simulink model "structure_lofi"  (R2026b)
settings: Solver=VariableStepAuto
undefined symbols (not defined in the file or in its folder): DiscIntNeverNeededParam, P, Ts
libraries: fl_lib x14, nesl_utility x10, simulink x5, robotmobilelib x1
settings Model: Creator=aomar  LastModifiedBy=aomar

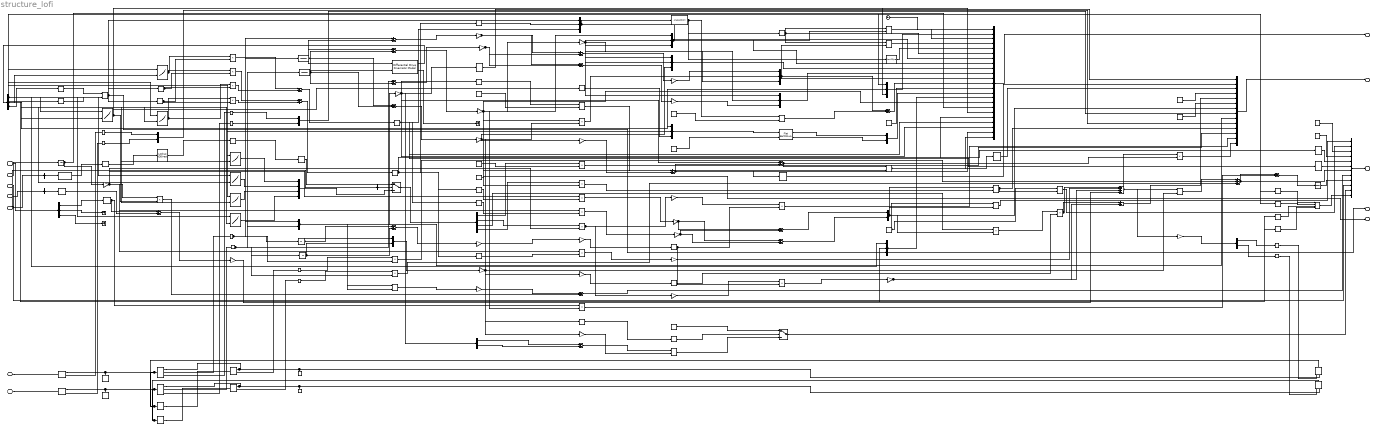
== system structure_lofi ==
  wrench : Inport
  dmdt : Inport  Port=2
  E_impl : Inport  Port=3
  env_dist : Inport  Port=4  OutDataTypeStr=Bus: Bus_EnvDisturbance
  env_ovr : Inport  Port=5  OutDataTypeStr=Bus: Bus_EnvOverride
  Br : Gain  Gain=P.structure.geom.B
  Clock : Clock
  DCM_WB : Angle2Dcm
      settings: AttributesFormatString=Rotation Order: %<rotationOrder>
  DDKM : robotmobilelib/Differential Drive Kinematic Model  VehicleInputs=Wheel Speeds  WheelRadius=P.structure.r_sprocket*(1-P.structure.lofi.i_nom)  WheelSpeedRange=[-inf inf]  TrackWidth=P.structure.lofi.chi*P.structure.geom.B  InitialState=P.structure.init.pose2D0(:)  SimulateUsing=Code generation
  D_R : UnaryMinus
  Dist : BusSelector  OutputSignals=F_ext_B
  E_diss_J : DiscreteIntegrator  gainval=1  SampleTime=Ts.base  ICPrevOutput=DiscIntNeverNeededParam  ICPrevScaledInput=DiscIntNeverNeededParam
  E_kin : Gain  Gain=0.5*P.structure.lofi.J_side
  E_mech : Sum
  E_pot : Product  Inputs=**
  F_diss : Sum
  F_grade : Gain  Gain=0.5
  F_load : Sum  Inputs=+++-
  F_push : Sum
  F_roll : Product  Inputs=**
  F_turn : Product  Inputs=**
  Fext_x : Selector  InputPortWidth=3  IndexOptions=Index vector (dialog)  Indices=1  OutputSizes=1
  Fimpl_x : Selector  InputPortWidth=3  IndexOptions=Index vector (dialog)  Indices=1  OutputSizes=1
  Flat_Earth_to_LLA : FlatEarth2LLA  LL0=P.world.lla0(1:2)
  Fric_Sensor_L : fl_lib/Mechanical/Mechanical Sensors/Ideal Torque Sensor
  Fric_Sensor_R : fl_lib/Mechanical/Mechanical Sensors/Ideal Torque Sensor
  Friction_L : fl_lib/Mechanical/Rotational Elements/Rotational Friction  brkwy_trq=P.structure.track.T_brk N*m  brkwy_vel=P.structure.track.w_brk rad/s  Col_trq=P.structure.track.T_col N*m  visc_coef=P.structure.track.c_visc N*m*s/rad  w_specify=off  w_priority=None  w=0 rad/s  w_nominal_specify=off  w_nominal_value=1  w_nominal_unit=rad/s  t_specify=off  t_priority=None  t=0 N*m  t_nominal_specify=off  t_nominal_value=1  t_nominal_unit=N*m
  Friction_R : fl_lib/Mechanical/Rotational Elements/Rotational Friction  brkwy_trq=P.structure.track.T_brk N*m  brkwy_vel=P.structure.track.w_brk rad/s  Col_trq=P.structure.track.T_col N*m  visc_coef=P.structure.track.c_visc N*m*s/rad  w_specify=off  w_priority=None  w=0 rad/s  w_nominal_specify=off  w_nominal_value=1  w_nominal_unit=rad/s  t_specify=off  t_priority=None  t=0 N*m  t_nominal_specify=off  t_nominal_value=1  t_nominal_unit=N*m
  H : Lookup_n-D  BreakpointsForDimension1=P.world.terrain.xE  BreakpointsForDimension2=P.world.terrain.yN  IndexSearchMethod=Evenly spaced points  Table=P.world.terrain.H  ExtrapMethod=Clip  InternalRulePriority=Speed  RndMeth=Simplest
      settings: InputPortMap=u0,u1
  J_side_L : fl_lib/Mechanical/Rotational Elements/Inertia  inertia=P.structure.lofi.J_side kg*m^2  num_ports=foundation.enum.numPorts2.one  w_specify=on  w_priority=High  w=P.structure.init.v0/P.structure.r_sprocket rad/s  w_nominal_specify=off  w_nominal_value=1  w_nominal_unit=rad/s  t_specify=off  t_priority=None  t=0 N*m  t_nominal_specify=off  t_nominal_value=1  t_nominal_unit=N*m
  J_side_R : fl_lib/Mechanical/Rotational Elements/Inertia  inertia=P.structure.lofi.J_side kg*m^2  num_ports=foundation.enum.numPorts2.one  w_specify=on  w_priority=High  w=P.structure.init.v0/P.structure.r_sprocket rad/s  w_nominal_specify=off  w_nominal_value=1  w_nominal_unit=rad/s  t_specify=off  t_priority=None  t=0 N*m  t_nominal_specify=off  t_nominal_value=1  t_nominal_unit=N*m
  Load_Torque_L : fl_lib/Mechanical/Mechanical Sources/Ideal Torque Source
  Load_Torque_R : fl_lib/Mechanical/Mechanical Sources/Ideal Torque Source
  Mass : Integrator  InitialCondition=P.structure.mp.m0
  Motion_Sensor_L : fl_lib/Mechanical/Mechanical Sensors/Ideal Rotational Motion Sensor  reference=foundation.enum.MeasurementReference.difference  acceleration_port=false  velocity_port=true  position_port=true  wrap_angle=false  offset=0 rad
  Motion_Sensor_R : fl_lib/Mechanical/Mechanical Sensors/Ideal Rotational Motion Sensor  reference=foundation.enum.MeasurementReference.difference  acceleration_port=false  velocity_port=true  position_port=true  wrap_angle=false  offset=0 rad
  Mres : Gain  Gain=-P.structure.geom.L/4
  Mturn : Product  Inputs=**
  N_L : Sum  Inputs=+-
  N_LR : Mux  Inputs=2
  N_R : Sum
  N_pt : Product  Inputs=**  Multiplication=Matrix(*)
  NaN : Constant  Value=NaN  VectorParams1D=off
  Ones2 : Constant  Value=ones(2,1)  VectorParams1D=off
  Out_of_map : Logic  Operator=OR  Inputs=4  AllPortsSameDT=off  OutDataTypeStr=boolean
  Ovr_soil_id : BusSelector  OutputSignals=soil_id
  Ovr_use_soil : BusSelector  OutputSignals=use_soil
  PSS_T_L : nesl_utility/PS-Simulink Converter  PhysicalDomain=network_engine_domain  SubClassName=ps_output  LeftPortType=input  RightPortType=output  PseudoPeriodic=off  Frequencies=[]  VectorFormat=inherit  Unit=N*m  AffineConversion=off
  PSS_T_R : nesl_utility/PS-Simulink Converter  PhysicalDomain=network_engine_domain  SubClassName=ps_output  LeftPortType=input  RightPortType=output  PseudoPeriodic=off  Frequencies=[]  VectorFormat=inherit  Unit=N*m  AffineConversion=off
  PSS_Tf_L : nesl_utility/PS-Simulink Converter  PhysicalDomain=network_engine_domain  SubClassName=ps_output  LeftPortType=input  RightPortType=output  PseudoPeriodic=off  Frequencies=[]  VectorFormat=inherit  Unit=N*m  AffineConversion=off
  PSS_Tf_R : nesl_utility/PS-Simulink Converter  PhysicalDomain=network_engine_domain  SubClassName=ps_output  LeftPortType=input  RightPortType=output  PseudoPeriodic=off  Frequencies=[]  VectorFormat=inherit  Unit=N*m  AffineConversion=off
  PSS_th_L : nesl_utility/PS-Simulink Converter  PhysicalDomain=network_engine_domain  SubClassName=ps_output  LeftPortType=input  RightPortType=output  PseudoPeriodic=off  Frequencies=[]  VectorFormat=inherit  Unit=rad  AffineConversion=off
  PSS_th_R : nesl_utility/PS-Simulink Converter  PhysicalDomain=network_engine_domain  SubClassName=ps_output  LeftPortType=input  RightPortType=output  PseudoPeriodic=off  Frequencies=[]  VectorFormat=inherit  Unit=rad  AffineConversion=off
  PSS_w_L : nesl_utility/PS-Simulink Converter  PhysicalDomain=network_engine_domain  SubClassName=ps_output  LeftPortType=input  RightPortType=output  PseudoPeriodic=off  Frequencies=[]  VectorFormat=inherit  Unit=rad/s  AffineConversion=off
  PSS_w_R : nesl_utility/PS-Simulink Converter  PhysicalDomain=network_engine_domain  SubClassName=ps_output  LeftPortType=input  RightPortType=output  PseudoPeriodic=off  Frequencies=[]  VectorFormat=inherit  Unit=rad/s  AffineConversion=off
  P_diss : Sum  Inputs=+++
  P_diss_E : Sum  Inputs=+-
  P_impl : Product  Inputs=**
  P_res : DotProduct  OutDataTypeStr=Inherit: Inherit via internal rule
  Pf_L : Product  Inputs=**
  Pf_R : Product  Inputs=**
  Pslip : Product  Inputs=**
  R_WB : Math  Operator=transpose
  Ref_L : fl_lib/Mechanical/Rotational Elements/Mechanical Rotational Reference
  Ref_R : fl_lib/Mechanical/Rotational Elements/Mechanical Rotational Reference
  SPS_load_L : nesl_utility/Simulink-PS Converter  PhysicalDomain=network_engine_domain  SubClassName=ps_input  LeftPortType=input  RightPortType=output  PseudoPeriodic=off  Frequencies=[]  NoiseDistribution=none  NoiseParameters=[]  Unit=N*m  AffineConversion=off  FilteringAndDerivatives=zero  SimscapeFilterOrder=1  InputFilterTimeConstant=0.001  UdotUserProvided=0
  SPS_load_R : nesl_utility/Simulink-PS Converter  PhysicalDomain=network_engine_domain  SubClassName=ps_input  LeftPortType=input  RightPortType=output  PseudoPeriodic=off  Frequencies=[]  NoiseDistribution=none  NoiseParameters=[]  Unit=N*m  AffineConversion=off  FilteringAndDerivatives=zero  SimscapeFilterOrder=1  InputFilterTimeConstant=0.001  UdotUserProvided=0
  Soil : Demux
  Soil_map : Mux
  Soil_props : Selector  InputPortWidth=6  IndexOptions=Index vector (dialog)  Indices=[2 4 5 6]  OutputSizes=1
  Soil_row : Reshape
  Soil_sw : Switch  Criteria=u2 ~= 0  SaturateOnIntegerOverflow=off  InputSameDT=off
  Soil_table : LookupNDDirect  InputsSelectThisObjectFromTable=Vector  Table=P.world.soilTable'  DiagnosticForOutOfRangeInput=None
  Spread : Constant  Value=kron(eye(2),ones(P.structure.track.Nc,1))  VectorParams1D=off
  State : Demux  Outputs=3
  StructureDiag : BusCreator  Inputs=12  OutDataTypeStr=Bus: Bus_StructureDiag  NonVirtualBus=on
  T_load : Gain  Gain=-P.structure.r_sprocket
  T_load_LR : Demux  Outputs=2
  Term_Mimpl : Terminator
  Term_rimpl : Terminator
  Term_stateDot : Terminator
  Torque_Sensor_L : fl_lib/Mechanical/Mechanical Sensors/Ideal Torque Sensor
  Torque_Sensor_R : fl_lib/Mechanical/Mechanical Sensors/Ideal Torque Sensor
  TrackState : BusCreator  Inputs=14  OutDataTypeStr=Bus: Bus_TrackState  NonVirtualBus=on
  TruthState : BusCreator  Inputs=23  OutDataTypeStr=Bus: Bus_TruthState  NonVirtualBus=on
  Wcos : Product  Inputs=**
  Weight : Gain  Gain=P.frames.g
  Wrench : Demux  Outputs=[3 3 3]
  Wsin_l : Product  Inputs=**
  Wsin_t : Product  Inputs=**
  Zero : Gain  Gain=0
  Zeros14a : Constant  Value=zeros(2*P.structure.track.Nc,1)  VectorParams1D=off
  Zeros14b : Constant  Value=zeros(2*P.structure.track.Nc,1)  VectorParams1D=off
  Zeros2a : Constant  Value=zeros(2,1)  VectorParams1D=off
  Zeros2b : Constant  Value=zeros(2,1)  VectorParams1D=off
  a_diff : Sum  Inputs=-+
  a_err_L : Sum  Inputs=+-
  a_err_R : Sum  Inputs=+-
  a_sum : Sum
  abs_r : Abs  ZeroCross=off  SaturateOnIntegerOverflow=off
  abs_vB : Abs  ZeroCross=off  SaturateOnIntegerOverflow=off
  acc_B : Mux  Inputs=3
  acc_W : Product  Inputs=**  Multiplication=Matrix(*)
  alpha_B : Mux  Inputs=3
  alpha_L : Gain  Gain=1/P.sim.ssc.tau_filt
  alpha_R : Gain  Gain=1/P.sim.ssc.tau_filt
  chi_eff : Switch  Criteria=u2 ~= 0  SaturateOnIntegerOverflow=off  InputSameDT=off
  chi_raw : Product  Inputs=*/
  cos_gl : Trigonometry  Operator=cos
  cos_psi : Trigonometry  Operator=cos
  cos_th : Trigonometry  Operator=cos
  dvB : Sum  Inputs=-+
  eul : Mux  Inputs=3
  fN : Product  Inputs=**
  fRoll_map : Lookup_n-D  BreakpointsForDimension1=P.world.terrain.xE  BreakpointsForDimension2=P.world.terrain.yN  IndexSearchMethod=Evenly spaced points  Table=P.world.soil.fRoll  ExtrapMethod=Clip  InternalRulePriority=Speed  RndMeth=Simplest
      settings: InputPortMap=u0,u1
  g_B : Product  Inputs=**  Multiplication=Matrix(*)
  g_enu : Constant  Value=[0;0;P.frames.g]  VectorParams1D=off
  grade_lat : Trigonometry  Operator=atan
  grade_long : Trigonometry  Operator=atan
  hE : Lookup_n-D  BreakpointsForDimension1=P.world.terrain.xE  BreakpointsForDimension2=P.world.terrain.yN  IndexSearchMethod=Evenly spaced points  Table=P.world.terrain.dHdE  ExtrapMethod=Clip  InternalRulePriority=Speed  RndMeth=Simplest
      settings: InputPortMap=u0,u1
  hE_c : Product  Inputs=**
  hE_s : Product  Inputs=**
  hN : Lookup_n-D  BreakpointsForDimension1=P.world.terrain.xE  BreakpointsForDimension2=P.world.terrain.yN  IndexSearchMethod=Evenly spaced points  Table=P.world.terrain.dHdN  ExtrapMethod=Clip  InternalRulePriority=Speed  RndMeth=Simplest
      settings: InputPortMap=u0,u1
  hN_c : Product  Inputs=**
  hN_s : Product  Inputs=**
  half : Gain  Gain=0.5
  half_B : Gain  Gain=[-1;1]*P.structure.geom.B/2
  half_push : Gain  Gain=0.5
  href : Constant  Value=-P.world.lla0(3)  VectorParams1D=off
  inv_vEps : Gain  Gain=1/P.structure.track.vEpsRR
  inv_wEps : Gain  Gain=1/P.structure.lofi.w_eps
  kN : Product  Inputs=**
  kNc : Constant  Value=P.structure.track.Nc*P.structure.contact.kc  VectorParams1D=off
  kScale_map : Lookup_n-D  BreakpointsForDimension1=P.world.terrain.xE  BreakpointsForDimension2=P.world.terrain.yN  IndexSearchMethod=Evenly spaced points  Table=P.world.soil.kScale  ExtrapMethod=Clip  InternalRulePriority=Speed  RndMeth=Simplest
      settings: InputPortMap=u0,u1
  k_lat : Gain  Gain=P.structure.lofi.h_cg/P.structure.geom.B
  k_turn : Gain  Gain=P.structure.geom.L/(4*P.structure.geom.B)
  kr : Gain  Gain=P.structure.r_sprocket*(1-P.structure.lofi.i_nom)/(P.structure.lofi.chi*P.structure.geom.B)
  kr_d : Gain  Gain=P.structure.r_sprocket*(1-P.structure.lofi.i_nom)/(P.structure.lofi.chi*P.structure.geom.B)
  krd : Gain  Gain=P.structure.r_sprocket*(1-P.structure.lofi.i_nom)/(P.structure.lofi.chi*P.structure.geom.B)
  kv : Gain  Gain=P.structure.r_sprocket*(1-P.structure.lofi.i_nom)/2
  kvd : Gain  Gain=P.structure.r_sprocket*(1-P.structure.lofi.i_nom)/2
  lla : Mux  Inputs=2
  muLat_map : Lookup_n-D  BreakpointsForDimension1=P.world.terrain.xE  BreakpointsForDimension2=P.world.terrain.yN  IndexSearchMethod=Evenly spaced points  Table=P.world.soil.muLat  ExtrapMethod=Clip  InternalRulePriority=Speed  RndMeth=Simplest
      settings: InputPortMap=u0,u1
  muPeak2 : Product  Inputs=**
  muPeak_map : Lookup_n-D  BreakpointsForDimension1=P.world.terrain.xE  BreakpointsForDimension2=P.world.terrain.yN  IndexSearchMethod=Evenly spaced points  Table=P.world.soil.muPeak  ExtrapMethod=Clip  InternalRulePriority=Speed  RndMeth=Simplest
      settings: InputPortMap=u0,u1
  muW : Product  Inputs=**
  omega_B : Mux  Inputs=3
  p_ned : Mux  Inputs=3
  pen_pt : Product  Inputs=**  Multiplication=Matrix(*)
  pos_W : Mux  Inputs=3
  pose2D_mux : Mux  Inputs=3
  psi : Trigonometry  Operator=atan2
  q_WB : Dcm2Quat
  r_cg_B : Constant  Value=P.structure.mp.rcg0_FLU(:)  VectorParams1D=off
  r_small : simulink/Logic and Bit Operations/Compare To Constant  relop=<  const=P.structure.track.chi_rmin  OutDataTypeStr=boolean
  sin_gl : Trigonometry
  sin_gt : Trigonometry
  sin_psi : Trigonometry
  sin_th : Trigonometry
  sink : Product  Inputs=*/
  slip : SignalConversion  OverrideOpt=off
  slip_LR : Product  Inputs=*/
  slopeLat : SignalConversion  OverrideOpt=off
  slopeLong : SignalConversion  OverrideOpt=off
  soil_dbl : DataTypeConversion  OutDataTypeStr=double  SaturateOnIntegerOverflow=off  RndMeth=Floor
  soil_idx0 : Bias  Bias=-1  SaturateOnIntegerOverflow=off
  specForce_B : Sum
  sprAngle : Mux  Inputs=2
  sprTorque : Mux  Inputs=2
  tan_lat : Sum  Inputs=-+
  tan_long : Sum
  tanh_r : Trigonometry  Operator=tanh
  tanh_vb : Trigonometry  Operator=tanh
  theta : UnaryMinus
  turn_sign : Gain  Gain=[-1;1]
  vB_floor : MinMax  Function=max  Inputs=2  ZeroCross=off
  vBelt : Gain  Gain=P.structure.r_sprocket
  vBelt_LR : Demux  Outputs=2
  vGround : Sum
  v_b_d : Gain  Gain=P.structure.r_sprocket
  v_belt : SignalConversion  OverrideOpt=off
  v_eps : Constant  Value=P.structure.track.v_eps_slip  VectorParams1D=off
  v_ground : SignalConversion  OverrideOpt=off
  v_r : Product  Inputs=**
  v_slip : Sum  Inputs=+-
  vel_B : Mux  Inputs=3
  vel_W : Product  Inputs=**  Multiplication=Matrix(*)
  w2J : DotProduct  OutDataTypeStr=Inherit: Inherit via internal rule
  w_d : Mux  Inputs=2
  w_delay_L : UnitDelay  InitialCondition=P.structure.init.v0/P.structure.r_sprocket  SampleTime=Ts.base
  w_delay_R : UnitDelay  InitialCondition=P.structure.init.v0/P.structure.r_sprocket  SampleTime=Ts.base
  w_diff : Sum  Inputs=-+
  w_filt_L : TransferFcn  Numerator=1  Denominator=[P.sim.ssc.tau_filt 1]
  w_filt_R : TransferFcn  Numerator=1  Denominator=[P.sim.ssc.tau_filt 1]
  w_raw : Mux  Inputs=2
  w_sum : Sum
  wd_diff : Sum  Inputs=-+
  x_hi : simulink/Logic and Bit Operations/Compare To Constant  relop=>  const=P.world.terrain.xE(end)  OutDataTypeStr=boolean
  x_lo : simulink/Logic and Bit Operations/Compare To Constant  relop=<  const=P.world.terrain.xE(1)  OutDataTypeStr=boolean
  y_hi : simulink/Logic and Bit Operations/Compare To Constant  relop=>  const=P.world.terrain.yN(end)  OutDataTypeStr=boolean
  y_lo : simulink/Logic and Bit Operations/Compare To Constant  relop=<  const=P.world.terrain.yN(1)  OutDataTypeStr=boolean
  Spr_L : PMIOPort  Side=Left  ConnectionType=Connection: foundation.mechanical.rotational.rotational
  Spr_R : PMIOPort  Port=2  Side=Left  ConnectionType=Connection: foundation.mechanical.rotational.rotational
  truth : Outport  OutDataTypeStr=Bus: Bus_TruthState
  tracks : Outport  Port=2  OutDataTypeStr=Bus: Bus_TrackState
  diag : Outport  Port=3  OutDataTypeStr=Bus: Bus_StructureDiag
  pose2D : Outport  Port=4
  speed_fwd : Outport  Port=5
  wires:
  wrench/1 -> Wrench/1  "wrench"
  dmdt/1 -> Mass/1  "dmdt"
  E_impl/1 -> StructureDiag/10  "E_impl_shaft_J"
  env_dist/1 -> Dist/1  "env_dist"
  env_ovr/1 -> Ovr_soil_id/1, Ovr_use_soil/1  "env_ovr"
  Ovr_soil_id/1 -> soil_dbl/1  "<soil_id>"
  Dist/1 -> Fext_x/1  "<F_ext_B>"
  Wrench/1 -> Fimpl_x/1  "F_impl"
  Wrench/2 -> Term_Mimpl/1  "M_impl"
  Wrench/3 -> Term_rimpl/1  "r_impl"
  sin_th/1 -> psi/1  "sin_th"
  cos_th/1 -> psi/2  "cos_th"
  Mass/1 -> TruthState/17, Weight/1  "mass"
  Fext_x/1 -> F_push/2  "Fext_x"
  soil_dbl/1 -> soil_idx0/1  "soil_dbl"
  PSS_T_L/1 -> sprTorque/1  "T_spr_L"
  PSS_T_R/1 -> sprTorque/2  "T_spr_R"
  psi/1 -> pose2D_mux/3, eul/1, cos_psi/1, sin_psi/1  "psi"
  soil_idx0/1 -> Soil_table/1  "soil_idx0"
  Weight/1 -> Wsin_l/1, muW/2, Wsin_t/1, E_pot/1, Wcos/1  "W"
  Fimpl_x/1 -> P_impl/1, F_push/1  "Fimpl_x"
  H/1 -> E_pot/2, D_R/1, pos_W/3, TruthState/18  "terrainH"
  sprTorque/1 -> TrackState/10  "sprTorque"
  F_push/1 -> half_push/1  "F_push"
  sin_psi/1 -> hE_s/2, hN_s/2  "sin_psi"
  E_pot/1 -> E_mech/2  "E_pot"
  cos_psi/1 -> hE_c/2, hN_c/2  "cos_psi"
  hE/1 -> hE_s/1, hE_c/1  "hE"
  hN/1 -> hN_c/1, hN_s/1  "hN"
  Soil_table/1 -> Soil_row/1  "Soil_table"
  PSS_th_L/1 -> sprAngle/1  "th_L"
  PSS_th_R/1 -> sprAngle/2  "th_R"
  PSS_w_L/1 -> a_err_L/1, w_filt_L/1, Pf_L/2, w_raw/1, w_delay_L/1  "w_L"
  PSS_w_R/1 -> w_filt_R/1, a_err_R/1, Pf_R/2, w_raw/2, w_delay_R/1  "w_R"
  hE_s/1 -> tan_lat/1  "hE_s"
  hE_c/1 -> tan_long/1  "hE_c"
  hN_c/1 -> tan_lat/2  "hN_c"
  hN_s/1 -> tan_long/2  "hN_s"
  Soil_row/1 -> Soil_props/1  "Soil_row"
  half_push/1 -> F_load/4  "F_push_side"
  muPeak_map/1 -> Soil_map/1  "muPeak"
  muLat_map/1 -> Soil_map/2  "muLat"
  fRoll_map/1 -> Soil_map/3  "fRoll"
  kScale_map/1 -> Soil_map/4  "kScale"
  sprAngle/1 -> TrackState/8  "sprAngle"
  Soil_map/1 -> Soil_sw/3  "soil_map"
  w_raw/1 -> vBelt/1, TrackState/9, w2J/2, w2J/1  "sprSpeed"
  PSS_Tf_L/1 -> Pf_L/1  "T_fric_L"
  PSS_Tf_R/1 -> Pf_R/1  "T_fric_R"
  tan_lat/1 -> grade_lat/1  "tan_lat"
  tan_long/1 -> grade_long/1  "tan_long"
  w_delay_L/1 -> wd_diff/1, w_d/1  "w_d_L"
  Soil_props/1 -> Soil_sw/1  "soil_ovr"
  w_delay_R/1 -> wd_diff/2, w_d/2  "w_d_R"
  w_filt_L/1 -> w_diff/1, a_err_L/2, w_sum/1, DDKM/1  "w_L"
  w_filt_R/1 -> w_diff/2, w_sum/2, a_err_R/2, DDKM/2  "w_R"
  Ovr_use_soil/1 -> Soil_sw/2  "<use_soil>"
  w_d/1 -> v_b_d/1  "w_d"
  a_err_L/1 -> alpha_L/1  "a_err_L"
  w_sum/1 -> kv/1  "w_sum"
  a_err_R/1 -> alpha_R/1  "a_err_R"
  w_diff/1 -> kr/1  "w_diff"
  wd_diff/1 -> kr_d/1  "wd_diff"
  grade_long/1 -> theta/1, sin_gl/1, TruthState/19, slopeLong/1, cos_gl/1  "grade_long"
  Pf_L/1 -> P_diss/2  "P_fric_L"
  Pf_R/1 -> P_diss/3  "P_fric_R"
  w2J/1 -> E_kin/1  "w2"
  grade_lat/1 -> eul/3, sin_gt/1, slopeLat/1, TruthState/20  "grade_lat"
  vBelt/1 -> vBelt_LR/1, v_slip/1, TruthState/21, v_belt/1, abs_vB/1  "vBelt_LR"
  Soil_sw/1 -> Soil/1  "soil"
  DDKM/1 -> State/1  "state"
  DDKM/2 -> Term_stateDot/1  "stateDot"
  Soil/1 -> muPeak2/1  "muPeak"
  Soil/2 -> muW/1  "muLat"
  Soil/3 -> fN/1  "fRoll"
  Soil/4 -> kN/1  "kScale"
  vBelt_LR/1 -> dvB/1  "vBelt_L"
  vBelt_LR/2 -> dvB/2  "vBelt_R"
  theta/1 -> eul/2  "theta"
  alpha_L/1 -> a_diff/1, a_sum/1  "alpha_L"
  abs_vB/1 -> vB_floor/1  "abs_vB"
  v_eps/1 -> vB_floor/2  "v_eps"
  kr/1 -> Br/1, abs_r/1, omega_B/3, v_r/2, half_B/1  "r"
  Ones2/1 -> muPeak2/2  "Ones2"
  kNc/1 -> kN/2  "kNc"
  cos_gl/1 -> Wcos/2  "cos_gl"
  sin_gt/1 -> Wsin_t/2  "sin_gt"
  kr_d/1 -> inv_wEps/1  "r_d"
  sin_gl/1 -> Wsin_l/2  "sin_gl"
  E_kin/1 -> E_mech/1  "E_kin"
  v_belt/1 -> TrackState/1  "v_belt"
  kv/1 -> P_impl/2, speed_fwd/1, vel_B/1, Zero/1, vGround/1, v_r/1, TruthState/16  "speed_fwd"
  alpha_R/1 -> a_diff/2, a_sum/2  "alpha_R"
  v_b_d/1 -> P_res/2, inv_vEps/1  "v_b_d"
  eul/1 -> TruthState/7, DCM_WB/1  "eul"
  a_sum/1 -> kvd/1  "a_sum"
  a_diff/1 -> krd/1  "a_diff"
  E_mech/1 -> StructureDiag/8  "E_mech"
  dvB/1 -> chi_raw/1  "dvB"
  Zero/1 -> alpha_B/2, alpha_B/1, acc_B/3, omega_B/2, omega_B/1, vel_B/3, vel_B/2  "Zero"
  D_R/1 -> p_ned/3  "D_R"
  vB_floor/1 -> slip_LR/2  "vB_floor"
  v_r/1 -> acc_B/2  "v_r"
  half_B/1 -> vGround/2  "rB2"
  muPeak2/1 -> TrackState/12  "muPeak"
  kN/1 -> sink/2  "k_track"
  Wcos/1 -> half/1  "Wcos"
  Wsin_t/1 -> k_lat/1  "Wsin_t"
  muW/1 -> k_turn/1, Mres/1  "muLat_W"
  inv_wEps/1 -> tanh_r/1  "inv_wEps"
  Wsin_l/1 -> F_grade/1  "Wsin_l"
  inv_vEps/1 -> tanh_vb/1  "inv_vEps"
  P_impl/1 -> P_diss_E/2  "P_impl_chassis"
  abs_r/1 -> r_small/1  "abs_r"
  Br/1 -> chi_raw/2  "B_r"
  vel_B/1 -> TruthState/8, vel_W/2  "vel_B"
  omega_B/1 -> TruthState/9  "omega_B"
  p_ned/1 -> Flat_Earth_to_LLA/1  "p_R_ned"
  vGround/1 -> TruthState/22, v_slip/2, v_ground/1  "vGround_LR"
  kvd/1 -> acc_B/1  "v_dot"
  krd/1 -> alpha_B/3  "r_dot"
  g_enu/1 -> g_B/2  "g_enu"
  href/1 -> Flat_Earth_to_LLA/2  "href"
  Mres/1 -> Mturn/1  "Mres"
  tanh_r/1 -> Mturn/2, F_turn/2  "tanh_r"
  F_grade/1 -> F_load/2  "F_grade"
  tanh_vb/1 -> F_roll/2  "tanh_vb"
  k_turn/1 -> F_turn/1  "k_turn"
  NaN/1 -> chi_eff/1  "NaN"
  r_small/1 -> chi_eff/2  "r_small"
  chi_raw/1 -> chi_eff/3  "chi_raw"
  half/1 -> N_R/1, N_L/1  "half"
  k_lat/1 -> N_R/2, N_L/2  "k_lat"
  DCM_WB/1 -> g_B/1, q_WB/1, R_WB/1  "R_BW"
  acc_B/1 -> specForce_B/1, acc_W/2, TruthState/11  "acc_B"
  alpha_B/1 -> TruthState/10  "alpha_B"
  v_slip/1 -> Pslip/2, slip_LR/1  "v_slip"
  N_L/1 -> N_LR/1  "N_L"
  N_R/1 -> N_LR/2  "N_R"
  R_WB/1 -> TruthState/6, acc_W/1, vel_W/1  "R_WB"
  g_B/1 -> specForce_B/2  "g_B"
  Mturn/1 -> TrackState/13  "Mturn"
  F_turn/1 -> turn_sign/1  "F_turn"
  v_ground/1 -> TrackState/2  "v_ground"
  chi_eff/1 -> StructureDiag/11  "chi_eff"
  Flat_Earth_to_LLA/1 -> lla/1  "mu_l"
  Flat_Earth_to_LLA/2 -> lla/2  "h_geo"
  pos_W/1 -> TruthState/2  "pos_W"
  lla/1 -> TruthState/14  "lla"
  pose2D_mux/1 -> TruthState/15, pose2D/1  "pose2D"
  N_LR/1 -> TrackState/7, sink/1, fN/2, N_pt/2  "Fn"
  Clock/1 -> TruthState/1  "t"
  specForce_B/1 -> TruthState/12  "specForce_B"
  vel_W/1 -> TruthState/3  "vel_W"
  acc_W/1 -> TruthState/4  "acc_W"
  r_cg_B/1 -> TruthState/13  "r_cg_B"
  slip_LR/1 -> TruthState/23, slip/1  "slip_LR"
  Spread/1 -> pen_pt/1, N_pt/1  "Spread"
  turn_sign/1 -> F_load/3, F_diss/2  "F_turn_LR"
  q_WB/1 -> TruthState/5  "q_WB"
  TruthState/1 -> truth/1  "truth"
  sink/1 -> TrackState/11, pen_pt/2  "sinkage"
  N_pt/1 -> StructureDiag/1  "N_pt"
  fN/1 -> F_roll/1  "fN"
  slip/1 -> TrackState/3  "slip"
  pen_pt/1 -> StructureDiag/2  "pen_pt"
  F_roll/1 -> F_load/1, F_diss/1  "F_roll"
  F_load/1 -> TrackState/5, T_load/1, Pslip/1  "Fx"
  F_diss/1 -> P_res/1  "F_diss"
  Zeros2a/1 -> TrackState/4  "s_shear"
  Zeros2b/1 -> TrackState/6  "Fy"
  Pslip/1 -> TrackState/14  "Pslip"
  P_res/1 -> P_diss/1  "P_res"
  T_load/1 -> T_load_LR/1  "minus_T_load"
  TrackState/1 -> tracks/1  "tracks"
  T_load_LR/1 -> SPS_load_L/1  "minus_T_load_L"
  T_load_LR/2 -> SPS_load_R/1  "minus_T_load_R"
  P_diss/1 -> StructureDiag/7, P_diss_E/1  "P_diss"
  P_diss_E/1 -> E_diss_J/1  "P_diss_E"
  x_lo/1 -> Out_of_map/1  "x_lo"
  x_hi/1 -> Out_of_map/2  "x_hi"
  y_lo/1 -> Out_of_map/3  "y_lo"
  y_hi/1 -> Out_of_map/4  "y_hi"
  Zeros14a/1 -> StructureDiag/3  "sX"
  Zeros14b/1 -> StructureDiag/4  "sY"
  Out_of_map/1 -> StructureDiag/12  "outOfMap"
  E_diss_J/1 -> StructureDiag/9  "E_diss_J"
  slopeLong/1 -> StructureDiag/5  "slopeLong"
  slopeLat/1 -> StructureDiag/6  "slopeLat"
  StructureDiag/1 -> diag/1  "diag"
  State/2 -> pose2D_mux/2, y_hi/1, kScale_map/2, y_lo/1, fRoll_map/2, muLat_map/2, muPeak_map/2, hE/2, p_ned/1, hN/2, H/2, pos_W/2  "y_N"
  State/1 -> pose2D_mux/1, kScale_map/1, x_hi/1, fRoll_map/1, x_lo/1, muLat_map/1, muPeak_map/1, p_ned/2, hE/1, hN/1, H/1, pos_W/1  "x_E"
  State/3 -> sin_th/1, cos_th/1  "theta"
  connections:
  Friction_L/RConn1 -- Fric_Sensor_L/LConn1
  Fric_Sensor_L/RConn1 -- Motion_Sensor_L/RConn1 -- Ref_L/LConn1 -- Load_Torque_L/RConn2
  PSS_Tf_L/LConn1 -- Fric_Sensor_L/RConn2
  Friction_R/RConn1 -- Fric_Sensor_R/LConn1
  Fric_Sensor_R/RConn1 -- Motion_Sensor_R/RConn1 -- Ref_R/LConn1 -- Load_Torque_R/RConn2
  PSS_Tf_R/LConn1 -- Fric_Sensor_R/RConn2
  J_side_L/LConn1 -- Torque_Sensor_L/RConn1 -- Motion_Sensor_L/LConn1 -- Friction_L/LConn1 -- Load_Torque_L/LConn1
  J_side_R/LConn1 -- Torque_Sensor_R/RConn1 -- Motion_Sensor_R/LConn1 -- Friction_R/LConn1 -- Load_Torque_R/LConn1
  SPS_load_L/RConn1 -- Load_Torque_L/RConn1
  SPS_load_R/RConn1 -- Load_Torque_R/RConn1
  PSS_w_L/LConn1 -- Motion_Sensor_L/RConn2
  PSS_th_L/LConn1 -- Motion_Sensor_L/RConn3
  PSS_w_R/LConn1 -- Motion_Sensor_R/RConn2
  PSS_th_R/LConn1 -- Motion_Sensor_R/RConn3
  PSS_T_L/LConn1 -- Torque_Sensor_L/RConn2
  PSS_T_R/LConn1 -- Torque_Sensor_R/RConn2
  Spr_L/RConn1 -- Torque_Sensor_L/LConn1
  Spr_R/RConn1 -- Torque_Sensor_R/LConn1
